simulink model "noiseModel"  (R2025b)
settings: Solver=FixedStepAuto  StartTime=0.0  StopTime=10  FixedStep=1e-5  RelTol=1e-3
undefined symbols (not defined in the file): noise
settings Model: Creator=pasqualederosa  LastModifiedBy=pasqualederosa

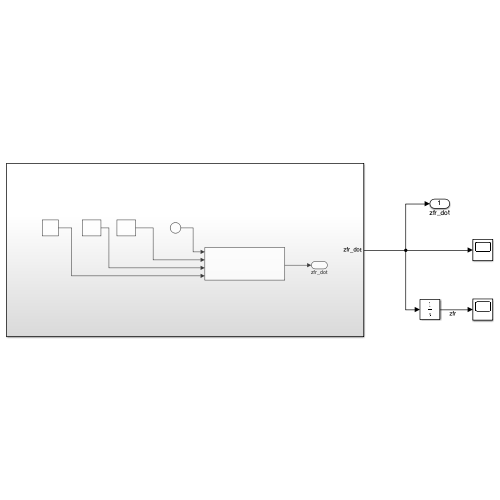
[thumbnail: Simulink's stored preview of the top-level diagram]
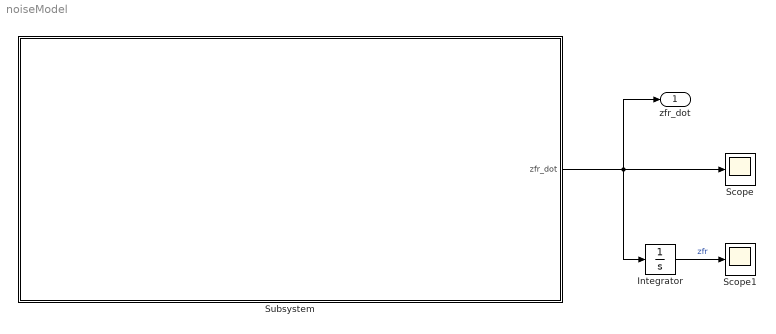
== system noiseModel ==
  Integrator : Integrator
  Scope : Scope
      settings: ActiveDisplayYMinimum=-0.062499999999999986  ActiveDisplayYMaximum=0.5625
  Scope1 : Scope
      settings: ActiveDisplayYMinimum=0.031249999997155404  ActiveDisplayYMaximum=0.031250000001234013
  Subsystem : Subsystem
  zfr_dot : Outport
  wires:
  Integrator/1 -> Scope1/1  "zfr"
  Subsystem/1(zfr_dot) -> Scope/1, zfr_dot/1, Integrator/1

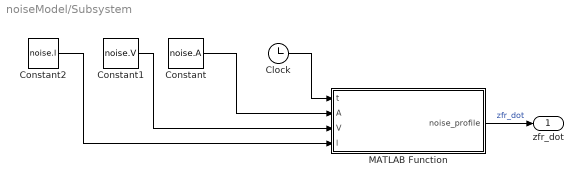
== system noiseModel/Subsystem ==
  Clock : Clock
  Constant : Constant  Value=noise.A
  Constant1 : Constant  Value=noise.V
  Constant2 : Constant  Value=noise.l
  MATLAB Function : MATLAB Function  TreatAsAtomicUnit=on
  zfr_dot : Outport
  wires:
  MATLAB Function/1(noise_profile) -> zfr_dot/1  "zfr_dot"
  Constant/1 -> MATLAB Function/2(A)
  Constant1/1 -> MATLAB Function/3(V)
  Constant2/1 -> MATLAB Function/4(l)
  Clock/1 -> MATLAB Function/1(t)

== matlab function noiseModel/Subsystem/MATLAB Function ==
  data: t input; noise_profile output; A input; V input; l input
function noise_profile = calc_noise(t, A, V, l)
    % This runs at every time step (no 'idx' or array looping needed)
    noise_profile = (A / 2) * (1 - cos((2 * pi * V / l) * t));
    if t>l/V
        noise_profile = 0;
    end
end
